simulink library "NEPTUN_MK"  (R2026a)
settings: Solver=VariableStepAuto
settings Model: Creator=Szalay  LastModifiedBy=Szalay

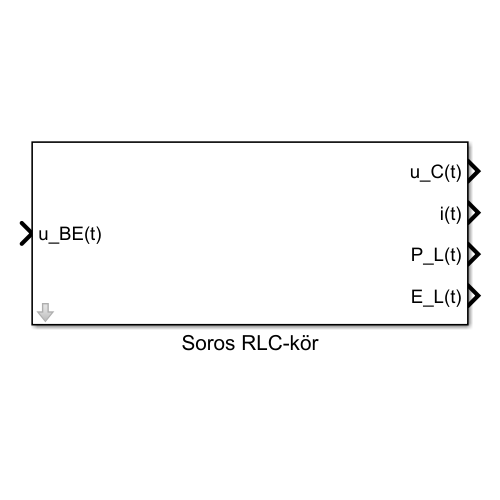
[thumbnail: Simulink's stored preview of the top-level diagram]
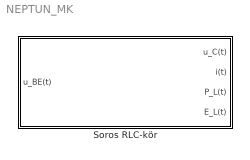
== system NEPTUN_MK ==
  Soros RLC-kör : Subsystem  mask(Soros RLC-kör){R=1, L=1e-3, tau=1, i_0=0, u_C0=0}
      mask prompts: R "Ellenállás"; L "Induktivitás"; tau "Időállandó"; i_0 "Kezdeti áramerősség"; u_C0 "Kezdeti kapacitás feszültség"
      mask help: A soros RLC-kör modellje.
      mask DialogControl ParameterGroupVar Prompt: Paraméterek
      mask DialogControl Container3 Prompt: Kezdeti értékek

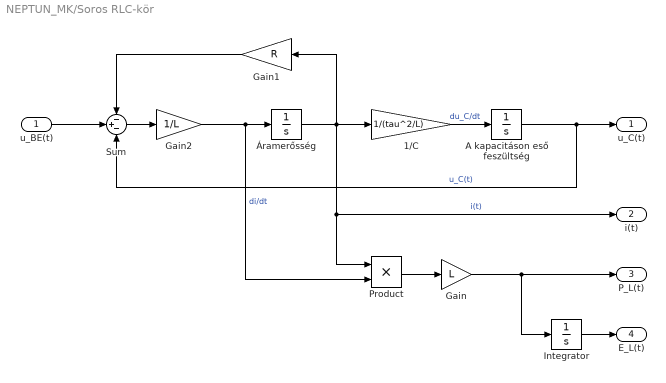
== system NEPTUN_MK/Soros RLC-kör ==
  u_BE(t) : Inport
  1/C : Gain  Gain=1/(tau^2/L)
  A kapacitáson eső feszültség : Integrator  InitialCondition=u_C0
  Gain : Gain  Gain=L
  Gain1 : Gain  Gain=R
  Gain2 : Gain  Gain=1/L
  Integrator : Integrator
  Product : Product
  Sum : Sum  Inputs=-+-
  Áramerősség : Integrator  InitialCondition=i_0
  u_C(t) : Outport
  i(t) : Outport  Port=2
  P_L(t) : Outport  Port=3
  E_L(t) : Outport  Port=4
  wires:
  1/C/1 -> A kapacitáson eső feszültség/1  "du_C/dt"
  Sum/1 -> Gain2/1
  Áramerősség/1 -> 1/C/1, Gain1/1, Product/1, i(t)/1  "i(t)"
  A kapacitáson eső feszültség/1 -> u_C(t)/1, Sum/3  "u_C(t)"
  u_BE(t)/1 -> Sum/2
  Gain2/1 -> Product/2, Áramerősség/1  "di/dt"
  Gain1/1 -> Sum/1
  Product/1 -> Gain/1
  Gain/1 -> Integrator/1, P_L(t)/1
  Integrator/1 -> E_L(t)/1
